simulink model "bsd"  (R2024a)
settings: Solver=FixedStepDiscrete  StartTime=0.0  StopTime=RIN_Stop_Time  FixedStep=RIN_Step_Size  RelTol=1e-3  EnableMultiTasking=on
undefined symbols (not defined in the file): D1, P
settings Model: DataDictionary=bsd.sldd  Creator=pc  LastModifiedBy=pc
settings SolverCC: AlgebraicLoopSolver=TrustRegion  PositivePriorityOrder=on  AutoInsertRateTranBlk=on  InsertRTBMode=Never (minimum delay)  MaxZcPerStep=1
settings OptimizationCC: DefaultParameterBehavior=Inlined  UseDivisionForNetSlopeComputation=on  GainParamInheritBuiltInType=on  UseFloatMulNetSlope=on  DefaultUnderspecifiedDataType=single  UseSpecifiedMinMax=on  InlineInvariantSignals=on  BitwiseOrLogicalOp=Bitwise operator  PassReuseOutputArgsAs=Individual arguments  ZeroExternalMemoryAtStartup=off  ZeroInternalMemoryAtStartup=off  NoFixptDivByZeroProtection=on  EfficientFloat2IntCast=on  LifeSpan=inf  MaxStackSize=64  OptimizeBlockOrder=speed  DifferentSizesBufferReuse=on  OptimizationLevel=level0  EfficientTunableParamExpr=on
settings DebuggingCC: SignalInfNanChecking=warning  ReadBeforeWriteMsg=EnableAllAsError  WriteAfterWriteMsg=EnableAllAsError  WriteAfterReadMsg=EnableAllAsError  IntegerOverflowMsg=error  ParameterTunabilityLossMsg=error  UnconnectedLineMsg=warning  UniqueDataStoreMsg=error  AssertControl=DisableAll  NonBusSignalsTreatedAsBus=error  SFInvalidInputDataAccessInChartInitDiag=error  SFTransitionOutsideNaturalParentDiag=error  SFUnreachableExecutionPathDiag=error  SFUndirectedBroadcastEventsDiag=error  IntegerSaturationMsg=error
settings HardwareCC: ProdBitPerPointer=32  ProdBitPerSizeT=32  ProdBitPerPtrDiffT=32  ProdLargestAtomicFloat=None  ProdWordSize=32  ProdLongLongMode=on  ProdHWDeviceType=Custom Processor->Custom Processor  HardwareBoardFeatureSet=SoCBlockset
settings ModelReferenceCC: EnableRefExpFcnMdlSchedulingChecks=on  ModelReferenceNumInstancesAllowed=Single
settings SFSimCC: CompileTimeRecursionLimit=0  EnableRuntimeRecursion=off  MATLABDynamicMemAlloc=off
settings RTWCC: Description=AUTOSAR  SystemTargetFile=autosar.tlc  GenCodeOnly=on  TemplateMakefile=ert_default_tmf  GenerateReport=on  CustomInclude=Rte_Type.h  BuildConfiguration=Faster Runs  IncludeHyperlinkInReport=on  LaunchReport=on  DataTypeReplacement=CDataTypesFixedWidth  GenerateWebview=on  CheckMdlBeforeBuild=Warning  GPUComputeCapability=3.5  DLArmComputeVersion=19.05
settings CodeAppCC: ForceParamTrailComments=on  IgnoreCustomStorageClasses=off  IgnoreTestpoints=on  OperatorAnnotations=on  SimulinkDataObjDesc=on  SFDataObjDesc=on  MATLABFcnDesc=on  InsertBlockDesc=on  ReqsInCode=on
settings STFCustomTargetCC: TargetLangStandard=C89/C90 (ANSI)  CodeReplacementLibrary=AUTOSAR 4.0  UtilityFuncGeneration=Shared location  MultiwordLength=256  ParMdlRefBuildCompliant=on  CompOptLevelCompliant=on  IncludeMdlTerminateFcn=off  CombineOutputUpdateFcns=on  CombineSignalStateStructs=on  SuppressErrorStatus=on  ERTCustomFileBanners=on  CodeInterfacePackaging=Reusable function  SupportNonFinite=off  SupportComplex=off  SupportContinuousTime=off  SupportNonInlinedSFcns=off  RemoveResetFunc=on  ParenthesesLevel=Standards  CastingMode=Standards  MATLABClassNameForMDSCustomization=Simulink.SoftwareTarget.ERTCustomization  AutosarCompliant=on  GRTInterface=off  GenerateSharedConstants=off  LookupTableObjectStructAxisOrder=2,1,3,4,...  LUTObjectStructOrderEvenSpacing=Size,Table,Breakpoints  SystemTargetFile=autosar.tlc
settings ERTTargetCC: CodeReplacementLibrary=AUTOSAR 4.0  UtilityFuncGeneration=Shared location  ConcurrentExecutionCompliant=off  IncludeMdlTerminateFcn=off  CombineSignalStateStructs=on  SuppressErrorStatus=on  CodeInterfacePackaging=Reusable function  SupportNonFinite=off  SupportComplex=off  ParenthesesLevel=Standards  CastingMode=Standards  ModelStepFunctionPrototypeControlCompliant=off  CPPClassGenCompliant=off  AutosarCompliant=on  GenerateSharedConstants=off  LookupTableObjectStructAxisOrder=2,1,3,4,...  LUTObjectStructOrderEvenSpacing=Size,Table,Breakpoints  ExtModeMexFile=noextcomm  InlinedParameterPlacement=NonHierarchical  ERTCustomFileTemplate=example_file_process.tlc  EnableSignedLeftShifts=off  EnableSignedRightShifts=off  BooleanTrueId=TRUE  BooleanFalseId=FALSE

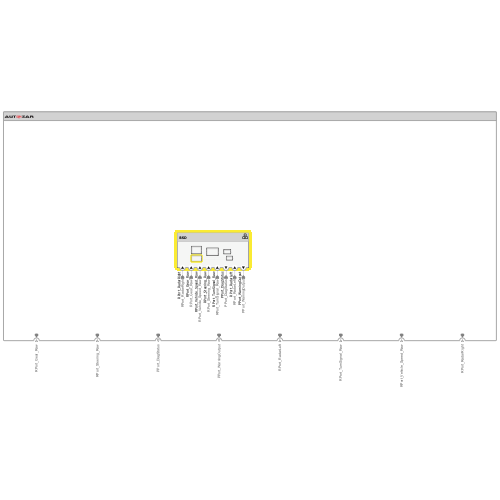
[thumbnail: Simulink's stored preview of the top-level diagram]
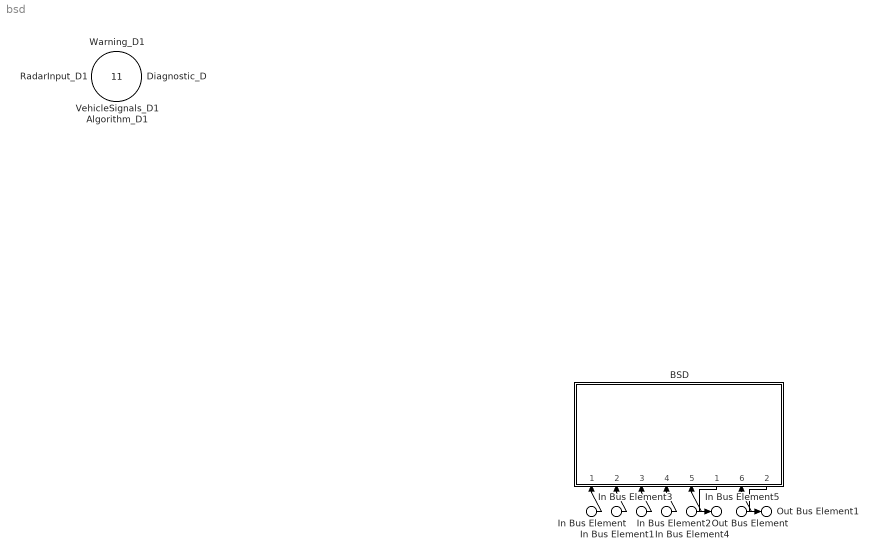
== system bsd ==
  In Bus Element : Inport  PortName=RPort_RadarRight
  In Bus Element1 : Inport  Port=2  PortName=RPort_Gear_Raw
  In Bus Element2 : Inport  Port=3  PortName=RPort_Vehicle_Speed_Raw
  In Bus Element3 : Inport  Port=4  PortName=RPort_Steering_Raw
  In Bus Element4 : Inport  Port=5  PortName=RPort_TurnSignal_Raw
  In Bus Element5 : Inport  Port=6  PortName=RPort_RadarLeft
  VehicleSignals_D1 : Inport  Port=7  OutputFunctionCall=on
  Warning_D1 : Inport  Port=8  OutputFunctionCall=on
  Algorithm_D1 : Inport  Port=9  OutputFunctionCall=on
  Diagnostic_D : Inport  Port=10  OutputFunctionCall=on
  RadarInput_D1 : Inport  Port=11  OutputFunctionCall=on
  BSD : Subsystem
      settings: PortSchema="{\"entries\":[{\"content\":{\"headerSize\":26,\"margin\":15,\"minimumSpacing\":25,\"sides\":[{\"content\":{},\"type\":\"ConnectorPlacement.EquallySpacedRectSide\",\"uuid\":\"6ee11bf0-3487-4de2-be00-6089215d7397\"},{\"content\":{\"side\":\"RIGHT\"},\"type\":\"ConnectorPlacement.EquallySpacedRectSide\",\"uuid\":\"80812468-7c6a-424f-b3e2-7cc7e0b0116a\"},{\"content\":{\"side\":\"TOP\"},\"type\":\"ConnectorPlacement.EquallySpacedRectSide\",\"uuid\":\"0bb877dd-8912-4ca5-a89b-901de1d19487\"},{\"content\":{\"connectorIds\":[\"In1\",\"In2\",\"In3\",\"In4\",\"In5\",\"Out1\",\"In6\",\"Out2\"],\"side\":\"BOTTOM\"},\"type\":\"ConnectorPlacement.EquallySpacedRectSide\",\"uuid\":\"d21e63ca-734c-4f62-8fe8-8baa088d181f\"}]},\"type\":\"ConnectorPlacement.EquallySpacedConnector\",\"uuid\":\"f31a2aac-102a-4ffb-961e-1f83b4d88391\"}],\"packageUris\":[\"http://schema.mathworks.com/mf0/Connector/R2020b\"],\"version\":\"1.0\"}"
  Out Bus Element : Outport  PortName=PPort_DiagStatus
  Out Bus Element1 : Outport  Port=2  PortName=PPort_WarningOutput
  wires:
  In Bus Element/1 -> BSD/1(RPort_RadarRight)
  In Bus Element1/1 -> BSD/2(RPort_Gear_Raw)
  In Bus Element2/1 -> BSD/3(RPort_Vehicle_Speed_Raw)
  In Bus Element3/1 -> BSD/4(RPort_Steering_Raw)
  In Bus Element4/1 -> BSD/5(RPort_TurnSignal_Raw)
  BSD/1(PPort_DiagStatus) -> Out Bus Element/1
  In Bus Element5/1 -> BSD/6(RPort_RadarLeft)
  BSD/2(PPort_WarningOutput) -> Out Bus Element1/1

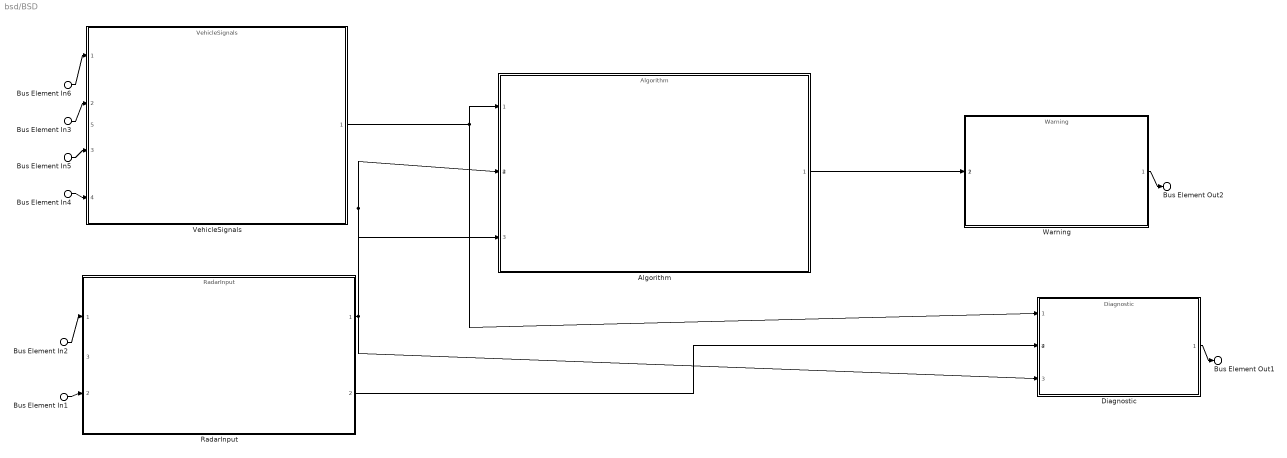
== system bsd/BSD ==
  Bus Element In2 : Inport  PortName=RPort_RadarRight
  Bus Element In4 : Inport  Port=2  PortName=RPort_Gear_Raw
  Bus Element In6 : Inport  Port=3  PortName=RPort_Vehicle_Speed_Raw
  Bus Element In5 : Inport  Port=4  PortName=RPort_Steering_Raw
  Bus Element In3 : Inport  Port=5  PortName=RPort_TurnSignal_Raw
  Bus Element In1 : Inport  Port=6  PortName=RPort_RadarLeft
  Algorithm : ModelReference  ModelNameDialog=Algorithm  SimulationMode=Normal  ScheduleRates=on  CachedPortDiscreteRates=[0.02]  ModelEventPortInfo=P:D1[0.02][0][0]  CodeInterface=Top model  ModelReferenceVersion=1.22
      settings: PortSchema="{\"entries\":[{\"content\":{\"headerSize\":38,\"margin\":15,\"minimumSpacing\":25,\"sides\":[{\"content\":{\"connectorIds\":[\"In1\",\"In2\",\"In3\"]},\"type\":\"ConnectorPlacement.EquallySpacedRectSide\",\"uuid\":\"6ee11bf0-3487-4de2-be00-6089215d7397\"},{\"content\":{\"connectorIds\":[\"Out1\"],\"side\":\"RIGHT\"},\"type\":\"ConnectorPlacement.EquallySpacedRectSide\",\"uuid\":\"80812468-7c6a-424f-b3e2-7cc7e0b0116a\"},{\"content\":{\"side\":\"TOP\"},\"type\":\"ConnectorPlacement.EquallySpacedRectSide\",\"uuid\":\"0bb877dd-8912-4ca5-a89b-901de1d19487\"},{\"content\":{\"connectorIds\":[\"In4\"],\"side\":\"HIDDEN\"},\"type\":\"ConnectorPlacement.EquallySpacedRectSide\",\"uuid\":\"a7058297-e58e-4c45-9731-5888b2c43cee\"}]},\"type\":\"ConnectorPlacement.EquallySpacedConnector\",\"uuid\":\"f31a2aac-102a-4ffb-961e-1f83b4d88391\"}],\"packageUris\":[\"http://schema.mathworks.com/mf0/Connector/R2020b\"],\"version\":\"1.0\"}"
  Diagnostic : ModelReference  ModelNameDialog=Diagnostic  SimulationMode=Normal  ScheduleRates=on  CachedPortDiscreteRates=[-1]  ModelEventPortInfo=P:D1[-1][0][0]  CodeInterface=Top model  ModelReferenceVersion=1.19
      settings: PortSchema="{\"entries\":[{\"content\":{\"headerSize\":38,\"margin\":15,\"minimumSpacing\":25,\"sides\":[{\"content\":{\"connectorIds\":[\"In1\",\"In2\",\"In3\"]},\"type\":\"ConnectorPlacement.EquallySpacedRectSide\",\"uuid\":\"6ee11bf0-3487-4de2-be00-6089215d7397\"},{\"content\":{\"connectorIds\":[\"Out1\"],\"side\":\"RIGHT\"},\"type\":\"ConnectorPlacement.EquallySpacedRectSide\",\"uuid\":\"80812468-7c6a-424f-b3e2-7cc7e0b0116a\"},{\"content\":{\"side\":\"TOP\"},\"type\":\"ConnectorPlacement.EquallySpacedRectSide\",\"uuid\":\"0bb877dd-8912-4ca5-a89b-901de1d19487\"},{\"content\":{\"connectorIds\":[\"In4\"],\"side\":\"HIDDEN\"},\"type\":\"ConnectorPlacement.EquallySpacedRectSide\",\"uuid\":\"c264ab3a-de67-4433-b40a-69376aaa21ff\"}]},\"type\":\"ConnectorPlacement.EquallySpacedConnector\",\"uuid\":\"f31a2aac-102a-4ffb-961e-1f83b4d88391\"}],\"packageUris\":[\"http://schema.mathworks.com/mf0/Connector/R2020b\"],\"version\":\"1.0\"}"
  RadarInput : ModelReference  ModelNameDialog=RadarInput  SimulationMode=Normal  ScheduleRates=on  CachedPortDiscreteRates=[0.02]  ModelEventPortInfo=P:D1[0.02][0][0]  CodeInterface=Top model  ModelReferenceVersion=1.87
      settings: PortSchema="{\"entries\":[{\"content\":{\"headerSize\":38,\"margin\":15,\"minimumSpacing\":25,\"sides\":[{\"content\":{\"connectorIds\":[\"In1\",\"In2\"]},\"type\":\"ConnectorPlacement.EquallySpacedRectSide\",\"uuid\":\"6ee11bf0-3487-4de2-be00-6089215d7397\"},{\"content\":{\"connectorIds\":[\"Out1\",\"Out2\"],\"side\":\"RIGHT\"},\"type\":\"ConnectorPlacement.EquallySpacedRectSide\",\"uuid\":\"80812468-7c6a-424f-b3e2-7cc7e0b0116a\"},{\"content\":{\"side\":\"TOP\"},\"type\":\"ConnectorPlacement.EquallySpacedRectSide\",\"uuid\":\"0bb877dd-8912-4ca5-a89b-901de1d19487\"},{\"content\":{\"side\":\"BOTTOM\"},\"type\":\"ConnectorPlacement.EquallySpacedRectSide\",\"uuid\":\"4a796927-7d0e-4bca-8bad-88887a703e86\"},{\"content\":{\"connectorIds\":[\"In3\"],\"side\":\"HIDDEN\"},\"type\":\"ConnectorPlacement.EquallySpacedRectSide\",\"uuid\":\"c1a32711-a242-4c56-ab78-ef4a6e58f5ea\"}]},\"type\":\"ConnectorPlacement.EquallySpacedConnector\",\"uuid\":\"f31a2aac-102a-4ffb-961e-1f83b4d88391\"}],\"packageUris\":[\"http://schema.mathworks.com/mf0/Connector/R2020b\"],\"version\":\"1.0\"}"
  VehicleSignals : ModelReference  ModelNameDialog=VehicleSignals  SimulationMode=Normal  ScheduleRates=on  CachedPortDiscreteRates=[0.02]  ModelEventPortInfo=P:D1[0.02][0][0]  CodeInterface=Top model  ModelReferenceVersion=1.61
      settings: PortSchema="{\"entries\":[{\"content\":{\"headerSize\":38,\"margin\":15,\"minimumSpacing\":25,\"sides\":[{\"content\":{\"connectorIds\":[\"In1\",\"In2\",\"In3\",\"In4\"]},\"type\":\"ConnectorPlacement.EquallySpacedRectSide\",\"uuid\":\"6ee11bf0-3487-4de2-be00-6089215d7397\"},{\"content\":{\"connectorIds\":[\"Out1\"],\"side\":\"RIGHT\"},\"type\":\"ConnectorPlacement.EquallySpacedRectSide\",\"uuid\":\"80812468-7c6a-424f-b3e2-7cc7e0b0116a\"},{\"content\":{\"side\":\"TOP\"},\"type\":\"ConnectorPlacement.EquallySpacedRectSide\",\"uuid\":\"0bb877dd-8912-4ca5-a89b-901de1d19487\"},{\"content\":{\"connectorIds\":[\"In5\"],\"side\":\"HIDDEN\"},\"type\":\"ConnectorPlacement.EquallySpacedRectSide\",\"uuid\":\"d41e763c-2317-4ad6-80f9-f1f661030115\"}]},\"type\":\"ConnectorPlacement.EquallySpacedConnector\",\"uuid\":\"f31a2aac-102a-4ffb-961e-1f83b4d88391\"}],\"packageUris\":[\"http://schema.mathworks.com/mf0/Connector/R2020b\"],\"version\":\"1.0\"}"
  Warning : ModelReference  ModelNameDialog=Warning  SimulationMode=Normal  ScheduleRates=on  CachedPortDiscreteRates=[0.02]  ModelEventPortInfo=P:D1[0.02][0][0]  CodeInterface=Top model  ModelReferenceVersion=1.12
      settings: PortSchema="{\"entries\":[{\"content\":{\"headerSize\":38,\"margin\":15,\"minimumSpacing\":25,\"sides\":[{\"content\":{\"connectorIds\":[\"In1\"]},\"type\":\"ConnectorPlacement.EquallySpacedRectSide\",\"uuid\":\"6ee11bf0-3487-4de2-be00-6089215d7397\"},{\"content\":{\"connectorIds\":[\"Out1\"],\"side\":\"RIGHT\"},\"type\":\"ConnectorPlacement.EquallySpacedRectSide\",\"uuid\":\"80812468-7c6a-424f-b3e2-7cc7e0b0116a\"},{\"content\":{\"side\":\"TOP\"},\"type\":\"ConnectorPlacement.EquallySpacedRectSide\",\"uuid\":\"0bb877dd-8912-4ca5-a89b-901de1d19487\"},{\"content\":{\"connectorIds\":[\"In2\"],\"side\":\"HIDDEN\"},\"type\":\"ConnectorPlacement.EquallySpacedRectSide\",\"uuid\":\"9069c7d9-0fc5-46e4-8315-c9f07adbffe8\"}]},\"type\":\"ConnectorPlacement.EquallySpacedConnector\",\"uuid\":\"f31a2aac-102a-4ffb-961e-1f83b4d88391\"}],\"packageUris\":[\"http://schema.mathworks.com/mf0/Connector/R2020b\"],\"version\":\"1.0\"}"
  Bus Element Out1 : Outport  PortName=PPort_DiagStatus
  Bus Element Out2 : Outport  Port=2  PortName=PPort_WarningOutput
  wires:
  Warning/1 -> Bus Element Out2/1
  Algorithm/1 -> Warning/1
  VehicleSignals/1 -> Algorithm/1, Diagnostic/1
  RadarInput/1 -> Algorithm/2, Algorithm/3, Diagnostic/3
  Bus Element In2/1 -> RadarInput/1
  Bus Element In1/1 -> RadarInput/2
  Diagnostic/1 -> Bus Element Out1/1
  Bus Element In4/1 -> VehicleSignals/4
  Bus Element In6/1 -> VehicleSignals/1
  Bus Element In3/1 -> VehicleSignals/2
  Bus Element In5/1 -> VehicleSignals/3
  RadarInput/2 -> Diagnostic/2
